simulink subsystem "dropper_trigger"  (R2026a)
settings: Solver=VariableStepAuto
undefined symbols (not defined in the file): S
libraries: ros2lib x2
PreSaveFcn:
  | defaultToFileBlockNames(bdroot);
settings Model: Creator=kjhaydon  LastModifiedBy=kjhaydon

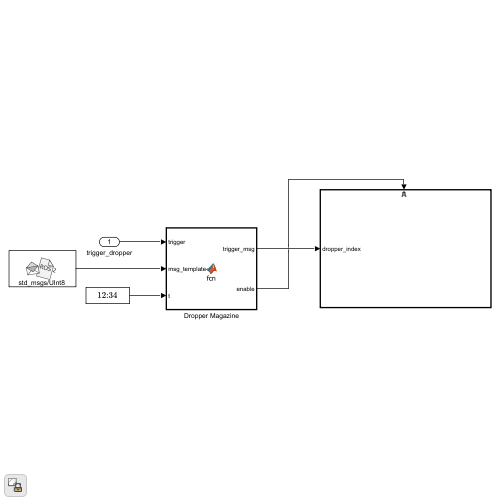
[thumbnail: Simulink's stored preview of the top-level diagram]
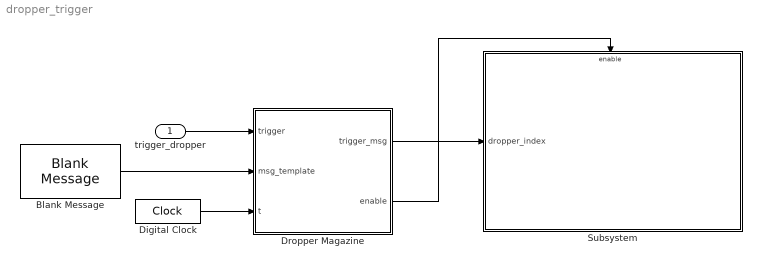
== system dropper_trigger ==
  trigger_dropper : Inport
  Blank Message : ros2lib/Blank Message  messageClass=Message  entityType=std_msgs/UInt8  messageType=std_msgs/UInt8  SampleTime=inf
  Digital Clock : DigitalClock  SampleTime=S.dt_control
  Dropper Magazine : MATLAB Function  TreatAsAtomicUnit=on
  Subsystem : Subsystem
  wires:
  trigger_dropper/1 -> Dropper Magazine/1(trigger)
  Dropper Magazine/2(enable) -> Subsystem/Enable
  Dropper Magazine/1(trigger_msg) -> Subsystem/1(dropper_index)
  Blank Message/1 -> Dropper Magazine/2(msg_template)
  Digital Clock/1 -> Dropper Magazine/3(t)

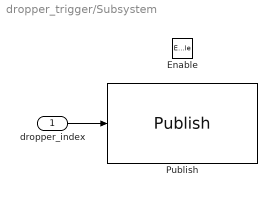
== system dropper_trigger/Subsystem ==
  dropper_index : Inport
  Enable : EnablePort
  Publish : ros2lib/Publish  topicSource=Specify your own  topic=/manipulator_cmd  messageType=std_msgs/UInt8  QOSHistory=Keep last  QOSDepth=10  QOSReliability=Reliable  QOSDurability=Volatile  QOSDeadline=Inf  QOSLifespan=Inf  QOSLiveliness=Automatic  QOSLeaseDuration=Inf  QOSAvoidROSNamespaceConventions=off
  wires:
  dropper_index/1 -> Publish/1

== matlab function dropper_trigger/Dropper Magazine ==
  data: trigger input; trigger_msg output Bus: SL_Bus_std_msgs_UInt8; msg_template input Bus: SL_Bus_std_msgs_UInt8; enable output; t input
function [trigger_msg, enable] = fcn(trigger, msg_template, t)

persistent ammo
persistent timeout
persistent last_drop_time

timeout_max = 1;

if(isempty(ammo))
    ammo = 2;
end
if(isempty(timeout))
    timeout = 0;
end
if(isempty(last_drop_time))
    last_drop_time = 0;
end

trigger_msg = msg_template;

if(t - last_drop_time > timeout_max)
    if(trigger && ammo > 0)
        trigger_msg.data = uint8(ammo);
        enable = true;
        ammo = ammo - 1;
        last_drop_time = t;
    else
        enable = false;
    end

else
    enable = false;

end
